simulink model "Engine_Torque"  (R2023b)
settings: Solver=VariableStepAuto  StartTime=0.0  StopTime=10.0  RelTol=1e-3
settings Model: Creator=leont  LastModifiedBy=leont

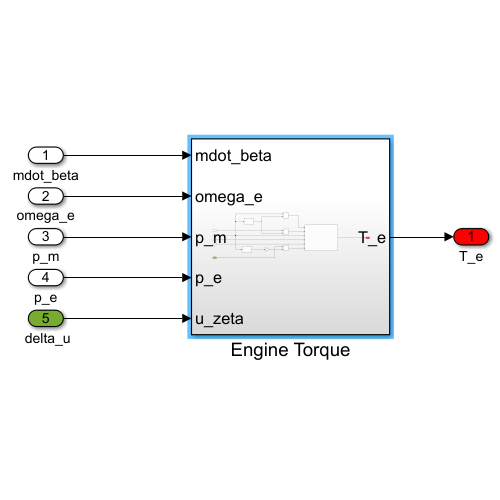
[thumbnail: Simulink's stored preview of the top-level diagram]
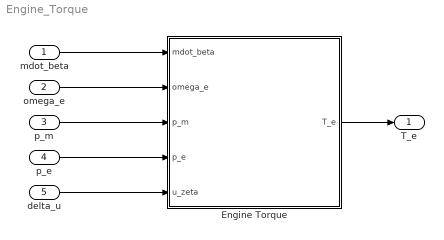
== system Engine_Torque ==
  mdot_beta : Inport
  omega_e : Inport  Port=2
  p_m : Inport  Port=3
  p_e : Inport  Port=4
  " delta_u" : Inport  Port=5
  Engine Torque : Subsystem
  T_e : Outport
  wires:
  mdot_beta/1 -> Engine Torque/1(mdot_beta)
  omega_e/1 -> Engine Torque/2(omega_e)
  p_m/1 -> Engine Torque/3(p_m)
  p_e/1 -> Engine Torque/4(p_e)
  " delta_u"/1 -> Engine Torque/5(u_zeta)
  Engine Torque/1(T_e) -> T_e/1

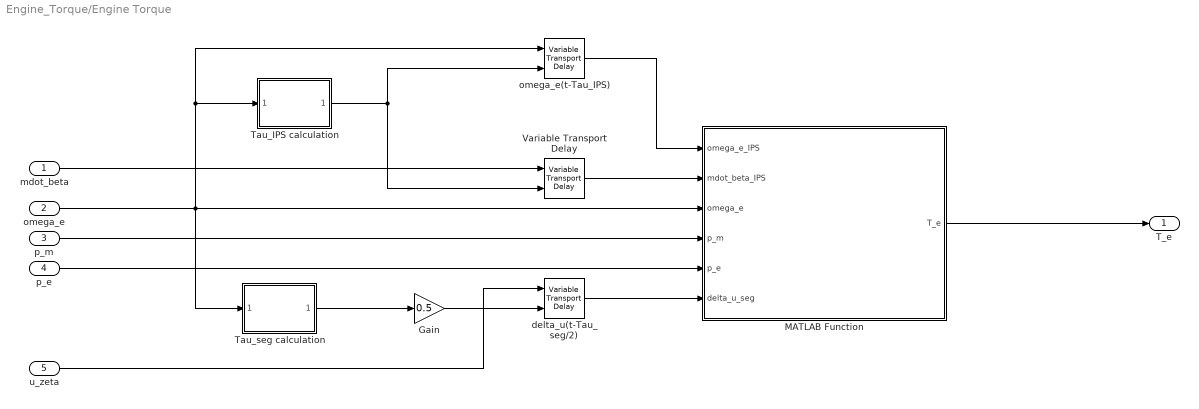
== system Engine_Torque/Engine Torque ==
  mdot_beta : Inport
  omega_e : Inport  Port=2
  p_m : Inport  Port=3
  p_e : Inport  Port=4
  u_zeta : Inport  Port=5
  Gain : Gain  Gain=0.5
  MATLAB Function : MATLAB Function  TreatAsAtomicUnit=on
  Tau_IPS calculation : MATLAB Function  TreatAsAtomicUnit=on
  Tau_seg calculation : MATLAB Function  TreatAsAtomicUnit=on
  Variable Transport Delay : VariableTransportDelay  MaximumDelay=10
  delta_u(t-Tau_seg/2) : VariableTransportDelay  MaximumDelay=10
  omega_e(t-Tau_IPS) : VariableTransportDelay  MaximumDelay=10
  T_e : Outport
  wires:
  Gain/1 -> delta_u(t-Tau_seg/2)/2
  p_m/1 -> MATLAB Function/4(p_m)
  omega_e/1 -> omega_e(t-Tau_IPS)/1, Tau_IPS calculation/1(omega_e), Tau_seg calculation/1(omega_e), MATLAB Function/3(omega_e)
  omega_e(t-Tau_IPS)/1 -> MATLAB Function/1(omega_e_IPS)
  Tau_IPS calculation/1(Tau_IPS) -> omega_e(t-Tau_IPS)/2, Variable Transport Delay/2
  Variable Transport Delay/1 -> MATLAB Function/2(mdot_beta_IPS)
  Tau_seg calculation/1(Tau_seg) -> Gain/1
  delta_u(t-Tau_seg/2)/1 -> MATLAB Function/6(delta_u_seg)
  u_zeta/1 -> delta_u(t-Tau_seg/2)/1
  MATLAB Function/1(T_e) -> T_e/1
  p_e/1 -> MATLAB Function/5(p_e)
  mdot_beta/1 -> Variable Transport Delay/1

== matlab function Engine_Torque/Engine Torque/Tau_IPS calculation ==
  data: omega_e input; Tau_IPS output
function Tau_IPS = fcn(omega_e)

    if omega_e > 0
        Tau_IPS = 2*pi/omega_e;
    
    else
        Tau_IPS = 0;
    end

end

== matlab function Engine_Torque/Engine Torque/MATLAB Function ==
  data: omega_e_IPS input; mdot_beta_IPS input; omega_e input; p_m input; p_e input; delta_u_seg input; T_e output
function T_e = fcn(omega_e_IPS, mdot_beta_IPS, omega_e, p_m, p_e, delta_u_seg)

%% Parameters to identify: beta0, eta0, eta1

p_me0f = beta0 * 4*pi/Vd;
p_me0g = p_e - p_m;
e_zeta = 1 - k_zeta*(delta_u_seg^2);
ep_mphi = (eta0 + eta1*omega_e)*e_zeta*Hl*4*pi*mdot_beta_IPS/(Vd*lamda*sigma0*omega_e_IPS);

p_me = (ep_mphi - p_me0f - p_me0g);


T_e = p_me*Vd/(4*pi);

== matlab function Engine_Torque/Engine Torque/Tau_seg calculation ==
  data: omega_e input; Tau_seg output
function Tau_seg = fcn(omega_e)

    if omega_e > 0
        Tau_seg = 4*pi/(5*omega_e);
    
    else
        Tau_seg = 0;
    end

end
